simulink model "CCCV_ICR18650"  (R2023b)
settings: Solver=ode23tb  StartTime=0.0  StopTime=10000  MaxStep=1  RelTol=1e-5  AbsTol=1e-7
model workspace (MAT data in the model file):
  Cth = 40.5
  Idis_plot = 0.95652
  Ilimit = 1.1
  Qrated = 2.2
  R0 = 0.016818
  Rth = 20
  SOC0 = [0 0 0 0]
  SOCstop = inf
  StopAtVoltage = 0
  Tamb = 25
  Tresponse = 10
  TsFIS = 1
  TsPower = 1
  Vcutoff = 4.2
  Vnom = 3.7
undefined symbols (not defined in the file or in its folder): Ion, Lithium
libraries: spsBatteryLib x4, spsBreakerLib x2, simulink x2, spsControlledCurrentSourceLib x1, spsControlledVoltageSourceLib x1, spsCurrentMeasurementLib x1, spsVoltageMeasurementLib x1, sps_lib x1
settings Model: Creator=LeoNick  LastModifiedBy=Leo Nick
settings DataIOCC: SaveOutput=off

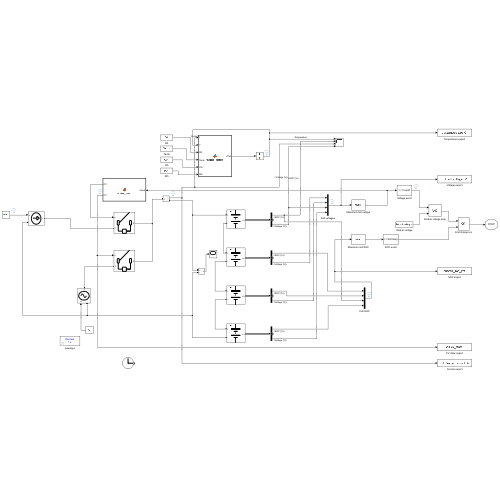
[thumbnail: Simulink's stored preview of the top-level diagram]
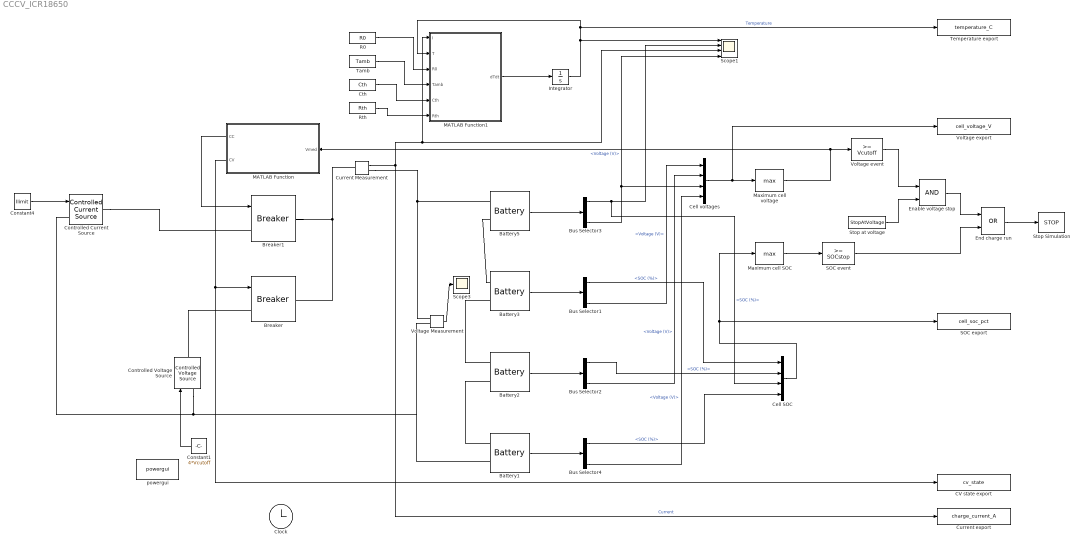
== system CCCV_ICR18650 ==
  Battery1 : spsBatteryLib/Battery  BatType=Lithium-Ion  ShowTempParam=off  ThermalPreset=no  ShowAgeParam=off  NomV=Vnom  NomQ=Qrated  SOC=SOC0(4)  Batt_Tr=Tresponse  PresetModel=on  MaxQ=2.2  MinV=2.775  FullV=4.3068  Dis_rate=0.95652  R=0.016818  Normal_OP=1.9896  expZone="[3.9974     0.10809]"  current=Idis_plot  Units=Time  Tci=20  NomT=20  T2=-30  MaxQ2=4.8  FullV2=7.1  Normal_OP2=5.655  expZone2="[6.58           1]"  Rca=0.6  ti=2000  Dp=0  Neq0=0  Tsim=1e6  Ta1=25  Qeol=5.4*0.9  Reol=0.013333*1.2  Char_age=[2.3478, 3]  Dis_age=[2.3478, 10]  N1=1500  N2=10500  N3=1000  N4=1400  Ta2=45  N5=950
  Battery2 : spsBatteryLib/Battery  BatType=Lithium-Ion  ShowTempParam=off  ThermalPreset=no  ShowAgeParam=off  NomV=Vnom  NomQ=Qrated  SOC=SOC0(2)  Batt_Tr=Tresponse  PresetModel=on  MaxQ=2.2  MinV=2.775  FullV=4.3068  Dis_rate=0.95652  R=0.016818  Normal_OP=1.9896  expZone="[3.9974     0.10809]"  current=Idis_plot  Units=Time  Tci=20  NomT=20  T2=-30  MaxQ2=4.8  FullV2=7.1  Normal_OP2=5.655  expZone2="[6.58           1]"  Rca=0.6  ti=2000  Dp=0  Neq0=0  Tsim=1e6  Ta1=25  Qeol=5.4*0.9  Reol=0.013333*1.2  Char_age=[2.3478, 3]  Dis_age=[2.3478, 10]  N1=1500  N2=10500  N3=1000  N4=1400  Ta2=45  N5=950
  Battery3 : spsBatteryLib/Battery  BatType=Lithium-Ion  ShowTempParam=off  ThermalPreset=no  ShowAgeParam=off  NomV=Vnom  NomQ=Qrated  SOC=SOC0(1)  Batt_Tr=Tresponse  PresetModel=on  MaxQ=2.2  MinV=2.775  FullV=4.3068  Dis_rate=0.95652  R=0.016818  Normal_OP=1.9896  expZone="[3.9974     0.10809]"  current=Idis_plot  Units=Time  Tci=20  NomT=20  T2=-30  MaxQ2=4.8  FullV2=7.1  Normal_OP2=5.655  expZone2="[6.58           1]"  Rca=0.6  ti=2000  Dp=0  Neq0=0  Tsim=1e6  Ta1=25  Qeol=5.4*0.9  Reol=0.013333*1.2  Char_age=[2.3478, 3]  Dis_age=[2.3478, 10]  N1=1500  N2=10500  N3=1000  N4=1400  Ta2=45  N5=950
  Battery5 : spsBatteryLib/Battery  BatType=Lithium-Ion  ShowTempParam=off  ThermalPreset=no  ShowAgeParam=off  NomV=Vnom  NomQ=Qrated  SOC=SOC0(3)  Batt_Tr=Tresponse  PresetModel=on  MaxQ=2.2  MinV=2.775  FullV=4.3068  Dis_rate=0.95652  R=0.016818  Normal_OP=1.9896  expZone="[3.9974     0.10809]"  current=Idis_plot  Units=Time  Tci=20  NomT=20  T2=-30  MaxQ2=4.8  FullV2=7.1  Normal_OP2=5.655  expZone2="[6.58           1]"  Rca=0.6  ti=2000  Dp=0  Neq0=0  Tsim=1e6  Ta1=25  Qeol=5.4*0.9  Reol=0.013333*1.2  Char_age=[2.3478, 3]  Dis_age=[2.3478, 10]  N1=1500  N2=10500  N3=1000  N4=1400  Ta2=45  N5=950
  Breaker : spsBreakerLib/Breaker  InitialState=0  SwitchingTimes="[1/60  5/60]"  External=on  BreakerResistance=0.01  SnubberResistance=1e6  SnubberCapacitance=inf  Measurements=None  MoreParameters=on  NoBreakLoop=off
  Breaker1 : spsBreakerLib/Breaker  InitialState=0  SwitchingTimes="[1/60  5/60]"  External=on  BreakerResistance=0.01  SnubberResistance=1e6  SnubberCapacitance=inf  Measurements=None  MoreParameters=on  NoBreakLoop=off
  Bus Selector{1..4} (4 alike) : BusSelector  OutputSignals=SOC (%),Current (A),Voltage (V)
  CV state export : ToWorkspace  VariableName=cv_state  SaveFormat=Timeseries  SampleTime=-1
  Cell SOC : Mux
  Cell voltages : Mux
  Clock : Clock
  Constant1 : Constant  Value=4*Vcutoff
  Constant4 : Constant  Value=Ilimit
  Controlled Current Source : spsControlledCurrentSourceLib/Controlled Current Source  Initialize=on  Source_Type=DC  Amplitude=0  Phase=0  Frequency=0  Measurements=None
  Controlled Voltage Source : spsControlledVoltageSourceLib/Controlled Voltage Source  Initialize=on  Source_Type=DC  Amplitude=0  Phase=0  Frequency=0  Measurements=None
  Cth : Constant  Value=Cth
  Current Measurement : spsCurrentMeasurementLib/Current Measurement  PhasorSimulation=off  OutputType=Complex  PSBequivalent=0
  Current export : ToWorkspace  VariableName=charge_current_A  SaveFormat=Timeseries  SampleTime=-1
  Enable voltage stop : Logic  AllPortsSameDT=off  OutDataTypeStr=boolean
  End charge run : Logic  Operator=OR  AllPortsSameDT=off  OutDataTypeStr=boolean
  Integrator : Integrator  InitialCondition=Tamb
  MATLAB Function : MATLAB Function  TreatAsAtomicUnit=on
  MATLAB Function1 : MATLAB Function  TreatAsAtomicUnit=on
  Maximum cell SOC : MinMax  Function=max
  Maximum cell voltage : MinMax  Function=max
  R0 : Constant  Value=R0
  Rth : Constant  Value=Rth
  SOC event : simulink/Logic and Bit Operations/Compare To Constant  relop=>=  const=SOCstop  OutDataTypeStr=boolean
  SOC export : ToWorkspace  VariableName=cell_soc_pct  SaveFormat=Timeseries  SampleTime=-1
  Scope1 : Scope  NumInputPorts=4
  Scope3 : Scope
  Stop Simulation : Stop
  Stop at voltage : Constant  Value=StopAtVoltage
  Tamb : Constant  Value=Tamb
  Temperature export : ToWorkspace  VariableName=temperature_C  SaveFormat=Timeseries  SampleTime=-1
  Voltage Measurement : spsVoltageMeasurementLib/Voltage Measurement  PhasorSimulation=off  OutputType=Complex  PSBequivalent=0
  Voltage event : simulink/Logic and Bit Operations/Compare To Constant  relop=>=  const=Vcutoff  OutDataTypeStr=boolean
  Voltage export : ToWorkspace  VariableName=cell_voltage_V  SaveFormat=Timeseries  SampleTime=-1
  powergui : sps_lib/powergui  Priority=1  SimulationMode=Discrete  SampleTime=TsPower  frequency=60  Iterations=50  frequencyindice=0  Pbase=100e6  ErrMax=1e-4  UnitsV=kV  UnitsW=MW  buscounter=0  FunctionMessages=off  echomessages=off  EnableUseOfTLC=off  CurrentSourceSwitches=off  DisableSnubberDevices=off  DisableRonSwitches=off  DisableVfSwitches=off  DisplayEquations=off  AutomaticDiscreteSolvers=off  SolverType=Tustin/Backward Euler (TBE)  Interpol=off  ExternalGateDelay=off  methode=off  Ts=100  x0status=blocks  SPID=on  SwTol=0  HookPort=off  NonlinearTolerance=1e-4  nMaxIteration=100  ContinueOnMaxIteration=off  RestoreLinks=warning  ResistiveCurrentMeasurement=off  Frange=[0:2:500]  Ylog=off  Xlog=on  ShowGrid=off  save=off  variable=ZData  structure=0  ZoomFFT=off  StartTime=0.0  cycles=1  DisplayStyle=1  fundamental=60  FreqAxis=off  MaxFrequency=1000  frequencyindicesteady=1  RmsSteady=1  display=off
  wires:
  Voltage Measurement/1 -> Scope3/1
  Battery1/1 -> Bus Selector4/1
  Bus Selector3/3 -> Scope1/4, Cell voltages/3  "<Voltage (V)>"
  Battery3/1 -> Bus Selector1/1
  Battery2/1 -> Bus Selector2/1
  Battery5/1 -> Bus Selector3/1
  MATLAB Function/1(CC) -> Breaker1/1
  MATLAB Function/2(CV) -> Breaker/1, CV state export/1
  Constant1/1 -> Controlled Voltage Source/1
  Constant4/1 -> Controlled Current Source/1
  Bus Selector3/1 -> Scope1/2, Cell SOC/3  "<SOC (%)>"
  Bus Selector1/1 -> Cell SOC/1  "<SOC (%)>"
  Bus Selector1/3 -> Cell voltages/1  "<Voltage (V)>"
  Bus Selector2/1 -> Cell SOC/2  "<SOC (%)>"
  Bus Selector2/3 -> Cell voltages/2  "<Voltage (V)>"
  Bus Selector4/1 -> Cell SOC/4  "<SOC (%)>"
  Bus Selector4/3 -> Cell voltages/4  "<Voltage (V)>"
  Current Measurement/1 -> Scope1/3, MATLAB Function1/1(I), Current export/1  "Current"
  MATLAB Function1/1(dTdt) -> Integrator/1
  Integrator/1 -> MATLAB Function1/2(T), Temperature export/1, Scope1/1  "Temperature"
  Cell voltages/1 -> Voltage export/1, Maximum cell voltage/1
  Cell SOC/1 -> Maximum cell SOC/1, SOC export/1
  Maximum cell voltage/1 -> MATLAB Function/1(Vmed), Voltage event/1
  Maximum cell SOC/1 -> SOC event/1
  Voltage event/1 -> Enable voltage stop/1
  Stop at voltage/1 -> Enable voltage stop/2
  Enable voltage stop/1 -> End charge run/1
  SOC event/1 -> End charge run/2
  End charge run/1 -> Stop Simulation/1
  R0/1 -> MATLAB Function1/3(R0)
  Tamb/1 -> MATLAB Function1/4(Tamb)
  Cth/1 -> MATLAB Function1/5(Cth)
  Rth/1 -> MATLAB Function1/6(Rth)
  connections:
  Breaker1/RConn1 -- Breaker/RConn1 -- Current Measurement/LConn1
  Battery1/LConn1 -- Battery2/LConn2
  Battery3/LConn2 -- Battery2/LConn1
  Battery5/LConn2 -- Battery3/LConn1
  Controlled Voltage Source/RConn1 -- Breaker/LConn1
  Controlled Voltage Source/LConn1 -- Battery1/LConn2 -- Voltage Measurement/LConn2 -- Controlled Current Source/LConn1
  Controlled Current Source/RConn1 -- Breaker1/LConn1
  Battery5/LConn1 -- Current Measurement/RConn1 -- Voltage Measurement/LConn1

== matlab function CCCV_ICR18650/MATLAB Function1 ==
  data: I input; dTdt output; T input; R0 input; Tamb input; Cth input; Rth input
function dTdt = modelo_termico(I,T,R0,Tamb,Cth,Rth)
dTdt = (I^2*R0 - (T-Tamb)/Rth)/Cth;
end

== matlab function CCCV_ICR18650/MATLAB Function ==
  data: Vmed input; CC output; CV output
function [CC, CV] = control_cccv(Vmed)

persistent estadoCV

% Inicialización
if isempty(estadoCV)
    estadoCV = false;
end

% Si todavía estamos en CC y se alcanza 4.2 V,
% cambiar permanentemente a CV
if ~estadoCV && Vmed >= 4.2
    estadoCV = true;
end

% Salidas hacia los conmutadores
if estadoCV
    CC = 0;
    CV = 1;
else
    CC = 1;
    CV = 0;
end

end
